simulink model "simulink_flightgear_control_trim_wind_5"  (R2023a)
settings: Solver=VariableStepAuto  StartTime=0  StopTime=inf  FixedStep=0.1  RelTol=1e-3
values from neighbouring files (symbols this model uses):
  model = 'simulink_flightgear_control_trim_wind_5'    [traimcode.m]
  ms2kts = 1.943844492609    (= 1.94384449261)    [Boeing747model.m]    (also in engine.m)
undefined symbols (not defined in the file or in its folder): Earth, F, Light, m, MIL, Model, Newton, Raphson, Receive, s, Send, Unit, WGS84, Wind
libraries: simulink_extras x7, aerolibconvert2 x5, simulink x4, aerolibfltsims x3, shared6dof x1, aerolibasang x1, aerolibtransform2 x1, aerolibatmos2 x1, aerolibobsolete x1, aerolibwind2 x1
(part 1 of 2)
settings Model: Creator=11759  LastModifiedBy=11759
settings SolverCC: ZeroCrossControl=DisableAll  ZeroCrossAlgorithm=Adaptive  EnableFixedStepZeroCrossing=on
settings DataIOCC: ExternalInput=getinputstruct(report2)  InitialState=getstatestruct(report2)  SaveFormat=StructureWithTime
settings OptimizationCC: BlockReduction=off  OptimizeBlockIOStorage=off  BufferReuse=off
settings DebuggingCC: AlgebraicLoopMsg=none  IgnoredZcDiagnostic=none
settings ModelReferenceCC: EnableRefExpFcnMdlSchedulingChecks=on
settings ExplorerConfigSet: SimMechanicsOpenEditorOnUpdate=off

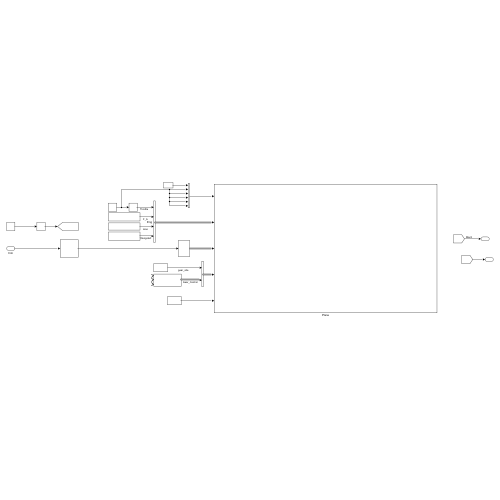
[thumbnail: Simulink's stored preview of the top-level diagram]
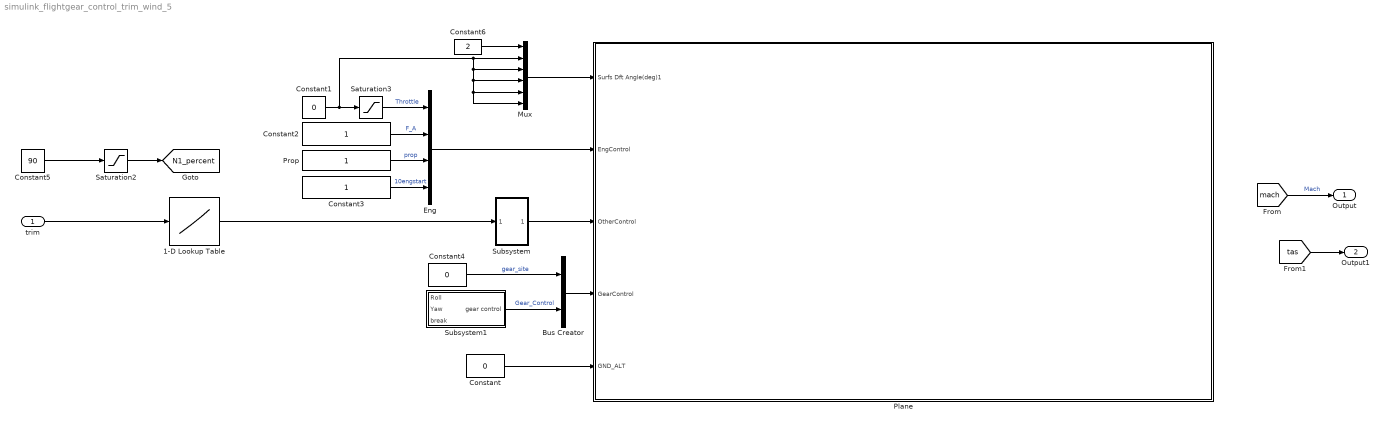
== system simulink_flightgear_control_trim_wind_5 ==
  trim : Inport
  1-D Lookup Table : Lookup_n-D  NumberOfTableDimensions=1  BreakpointsForDimension1=[-1 0 1]  Table=[-10 0 10]  InternalRulePriority=Speed  RndMeth=Simplest
  Bus Creator : BusCreator  Inputs=2
  Constant : Constant  Value=0
  Constant1 : Constant  Value=0
  Constant2 : Constant
  Constant3 : Constant
  Constant4 : Constant  Value=0
  Constant5 : Constant  Value=90
  Constant6 : Constant  Value=2
  Eng : BusCreator  Inputs=4
  Mux : Mux  Inputs=6
  Plane : Subsystem
      mask Display: image('$imagefile'); % 使用工具条上的 "编辑图像" 进行更改。
  Prop : Constant
  Saturation2 : Saturate  UpperLimit=110  LowerLimit=60
  Saturation3 : Saturate  UpperLimit=1  LowerLimit=0
  Subsystem : Subsystem
  Subsystem1 : Subsystem
  Output : Outport
  Output1 : Outport  Port=2
  tag scope: N1_percent=global
  wires:
  Mux/1 -> Plane/1(Surfs Dft Angle(deg)1)
  Constant/1 -> Plane/5(GND_ALT)
  Constant1/1 -> Mux/6, Mux/5, Mux/4, Mux/3, Mux/2, Saturation3/1
  Subsystem/1(Out1) -> Plane/3(OtherControl)
  Constant3/1 -> Eng/4  "10engstart"
  Prop/1 -> Eng/3  "prop"
  Subsystem1/1(gear control) -> Bus Creator/2  "Gear_Control"
  Constant2/1 -> Eng/2  "F_A"
  Saturation3/1 -> Eng/1  "Throttle"
  Eng/1 -> Plane/2(EngControl)
  Constant4/1 -> Bus Creator/1  "gear_site"
  Bus Creator/1 -> Plane/4(GearControl)
  Constant6/1 -> Mux/1
  Saturation2/1 -> [N1_percent]
  trim/1 -> 1-D Lookup Table/1
  1-D Lookup Table/1 -> Subsystem/1(In1)
  Constant5/1 -> Saturation2/1
  [mach] -> Output/1  "Mach"
  [tas] -> Output1/1

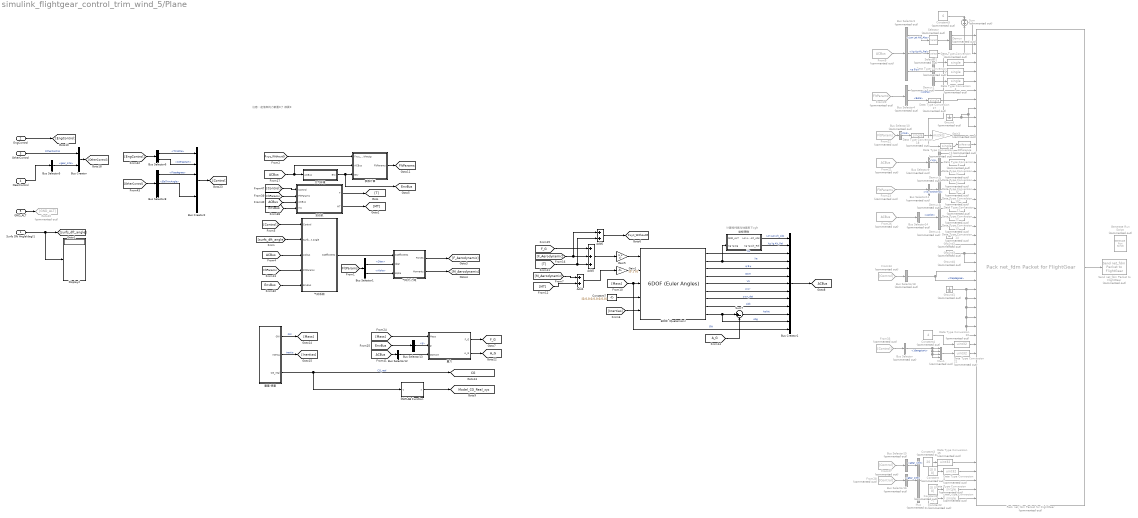
== system simulink_flightgear_control_trim_wind_5/Plane ==
  note: 注意：起落架的力都置0了
      | 襟翼0
  note: 计算经纬高与地面系下xyh
  Surfs Dft Angle(deg)1 : Inport
  EngControl : Inport  Port=2
  OtherControl : Inport  Port=3
  GearControl : Inport  Port=4
  GND_ALT : Inport  Port=5
  6DOF (Quaternion) : shared6dof/6DOF (Euler Angles)  units=Metric (MKS)  mtype=Custom Variable  rep=Euler Angles  xme_0=[0, 0, -Model.Init.Alt_Abs]  Vm_0=[Model.Init.u, Model.Init.v, Model.Init.w]  eul_0=[Model.Init.Roll, Model.Init.Pitch, Model.Init.Heading]  pm_0=[Model.Init.p, Model.Init.q, Model.Init.r]  mass_0=model.mass  mass_e=0  mass_f=0  inertia=[model.Ix -model.Ixy -model.Izx; -model.Ixy model.Iy -model.Iyz; -model.Izx -model.Iyz model.Iz]  inertia_e=eye(3)  inertia_f=eye(3)  k_quat=1.0  vre_flag=off  abi_flag=on  aMode=aMode  xme_statename=''  Vm_statename=''  eul_statename=''  quat_statename=''  pm_statename=''  mass_statename=''
  Add4 : Sum
  Add5 : Sum  Inputs=+++
  Add6 : Sum
  Bus Creator : BusCreator  Inputs=2
  Bus Creator1 : BusCreator  Inputs=13
  Bus Creator2 : BusCreator  Inputs=6
  Bus Selector : BusSelector  Commented=on  OutputSignals=10engstart
  Bus Selector1 : BusSelector  OutputSignals=Qbar,Alpha
  Bus Selector10 : BusSelector  Commented=on  OutputSignals=CAS
  Bus Selector11 : BusSelector  Commented=on  OutputSignals=Vb_WithWind
  Bus Selector12 : BusSelector  OutputSignals=DCM  OutputAsBus=on
  Bus Selector13 : BusSelector  OutputSignals=g
  Bus Selector14 : BusSelector  Commented=on  OutputSignals=Apilot
  Bus Selector15 : BusSelector  Commented=on  OutputSignals=gear_site
  Bus Selector16 : BusSelector  Commented=on  OutputSignals=gear_site
  Bus Selector18 : BusSelector  Commented=on  OutputSignals=Flapdegree
  Bus Selector3 : BusSelector  Commented=on  OutputSignals=Lon Lat Alt_Abs,Xg Yg Alt_Rel,φ θ ψ
  Bus Selector4 : BusSelector  Commented=on  OutputSignals=Alpha,Beta
  Bus Selector5 : BusSelector  OutputSignals=gear_site
  Bus Selector6 : BusSelector  OutputSignals=Throttle,10engstart
  Bus Selector8 : BusSelector  OutputSignals=OtherControl.Flapdegree,OtherControl.EleTrimAngle,OtherControl.SpoilerPercent
  Bus Selector9 : BusSelector  Commented=on  OutputSignals=Vg
  Constant : Constant  Commented=on  Value=[0 0 0]
  Constant1 : Constant  Commented=on  Value=[0 0 0]
  Constant2 : Constant  Commented=on  Value=[0 0 0]
  Constant3 : Constant  Commented=on  Value=20
  Constant4 : Constant  Commented=on  Value=4
  Constant5 : Constant  Commented=on  Value=6
  Constant7 : Constant  Value=[0,0,0;0,0,0;0,0,0]
  Data Type Conversion{,1..7,9..14,17..19} (17 alike) : DataTypeConversion  Commented=on  OutDataTypeStr=single  SaturateOnIntegerOverflow=off  RndMeth=Floor
  Data Type Conversion{8,15,20..21} (4 alike) : DataTypeConversion  Commented=on  OutDataTypeStr=uint32  SaturateOnIntegerOverflow=off  RndMeth=Floor
  Demux : Demux  Commented=on  Outputs=2
  Demux{1..4} (4 alike) : Demux  Commented=on  Outputs=3
  Difference : simulink/Discrete/Difference  Commented=on  ICPrevInput=0.0  OutMin=[]  OutMax=[]  OutDataType=fixdt(1, 16)  OutScaling=2^-10  DoSatur=off
  Display2 : Display
  From20 : From  Commented=on  GotoTag=FltParams  TagVisibility=global
  From21 : From  Commented=on  GotoTag=ACBus  TagVisibility=global
  From22 : From  Commented=on  GotoTag=FltParams  TagVisibility=global
  From23 : From  Commented=on  GotoTag=FltParams  TagVisibility=global
  From26 : From  Commented=on  GotoTag=ACBus  TagVisibility=global
  From{27..28,33..34} (4 alike) : From  Commented=on  GotoTag=Control
  From9 : From  Commented=on  GotoTag=ACBus  TagVisibility=global
  Gain1 : Gain  Gain=[0 1 0]'
  Gain3 : Gain  Commented=on  Gain=ms2kts
  Gain5 : Gain  Gain=[1 0 1]'
  Generate Run Script : aerolibfltsims/Generate Run Script  Commented=on  Architecture=Win64  dataFlow=Send-Receive  GeometryModelName=747-400  AirportId=KSFO  RunwayId=10L  InitialAltitude=1000  InitialHeading=113  OffsetDistance=4.72  OffsetAzimuth=0  InstallScenery=off  DisableShaders=on  OriginAddress=127.0.0.1  DestinationPort=5502  OriginPort=5505  LocalAddress=127.0.0.1  OutputFileName=runfg.bat  FlightGearBaseDirectory=E:\flightgear\FlightGear 2020.3
  Goto20 : Goto  Commented=on  GotoTag=GND_ALT
  Ground{,1..4} (5 alike) : Ground  Commented=on
  MATLAB Function : MATLAB Function  TreatAsAtomicUnit=on
  Mux : Mux  Commented=on  Inputs=3
  Mux1 : Mux  Commented=on
  Pack net_fdm Packet for FlightGear : aerolibfltsims/Pack net_fdm Packet for FlightGear  Commented=on  FlightGearVersion=v2019.1  ShowPositionAttitudeInputs=on  ShowVelocityAccelerationInputs=on  ShowControlSurfacePositionInputs=on  ShowEngineFuelInputs=on  ShowLandingGearInputs=on  ShowEnvironmentInputs=off  SampleTime=0.1  packetVersion=24
  Selector : Selector  Commented=on  InputPortWidth=3  IndexOptions=Index vector (dialog)  Indices=[1 2]  OutputSizes=1
  Selector1 : Selector  Commented=on  InputPortWidth=3  IndexOptions=Index vector (dialog)  Indices=[3]  OutputSizes=1
  Send net_fdm Packet to FlightGear : aerolibfltsims/Send net_fdm Packet to FlightGear  Commented=on  DestinationIpAddress=127.0.0.1  DestinationPort=5502  LocalIpPort=-1  varLen=off  SampleTime=0.1
  Sum : Sum  Commented=on
  Sum7 : Sum  Inputs=|+-
  参数计算 : Subsystem
  发动机 : Subsystem
  坐标转换 : Subsystem
  大气环境 : Subsystem
  气动力/力矩 : Subsystem
  气动系数 : Subsystem
  "重力 " : Subsystem
  重量/惯量 : Subsystem
  tag scope: ACBus=global, A_G=global, CG=global, EnvBus=global, F_G=global, FltParams=global, Fxyz_WithoutG=global, Model_CG_Real_xyz=global
  wires:
  EngControl/1 -> [EngControl]
  OtherControl/1 -> Bus Creator/1  "OtherControl"
  Bus Creator/1 -> [OtherControl]
  GearControl/1 -> Bus Selector5/1
  Bus Selector5/1 -> Bus Creator/2  "<gear_site>"
  GND_ALT/1 -> Goto20/1
  Bus Selector6/1 -> Bus Creator2/1  "<Throttle>"
  Bus Creator2/1 -> [Control]
  Bus Selector8/1 -> Bus Creator2/3  "<Flapdegree>"
  Bus Selector6/2 -> Bus Creator2/2  "<10engstart>"
  [EngControl] -> Bus Selector6/1
  [OtherControl] -> Bus Selector8/1
  Surfs Dft Angle(deg)1/1 -> [surfs_dft_angle], Display2/1
  [ACBus] -> 气动系数/3(ACbus)
  [Control] -> 气动系数/1(Control)
  [FltParams] -> 气动系数/4(FltParams)
  [surfs_dft_angle] -> 气动系数/2(Surfs Dft Angle)
  Bus Selector8/2 -> Bus Creator2/5  "<EleTrimAngle>"
  [EnvBus] -> 气动系数/5(EnvBus)
  MATLAB Function/1(y) -> [Model_CG_Real_xyz]
  重量/惯量/3(CG_real) -> MATLAB Function/1(u), [CG]  "CG_real"
  重量/惯量/1(GW) -> [Mass]  "GW"
  重量/惯量/2(Inertia) -> [Inertias]  "Inertia"
  发动机/1(T) -> [T]
  [ACBus] -> 发动机/3(ACBus)
  [Control] -> 发动机/1(Control)
  [ACBus] -> 大气环境/1(ACBus), 参数计算/2(ACBus)
  [EnvBus] -> 发动机/4(In1)
  大气环境/1(Env) -> [EnvBus], 参数计算/3(Env)
  [Fxyz_WithoutG] -> 参数计算/1(Fxyz_withoutg)
  发动机/2(MT) -> [MT]
  参数计算/1(FltParams) -> [FltParams]
  [FltParams] -> 发动机/2(FltParams)
  [FltParams] -> Bus Selector1/1
  Bus Selector1/1 -> 气动力/力矩/2(qbar)  "<Qbar>"
  Bus Selector1/2 -> 气动力/力矩/3(alpha)  "<Alpha>"
  气动系数/1(Coefficients) -> 气动力/力矩/1(Coefficients)
  气动力/力矩/2(Moments) -> [M_Aerodynamic]
  气动力/力矩/1(Forces) -> [F_Aerodynamic]
  "重力 "/1(F_G) -> [F_G]
  Bus Selector13/1 -> "重力 "/2(g)  "<g>"
  [EnvBus] -> Bus Selector13/1
  Bus Selector12/1 -> "重力 "/3(DCMwe)
  [ACBus] -> Bus Selector12/1
  [Mass] -> "重力 "/1(Mass)
  "重力 "/2(A_G) -> [A_G]
  Bus Selector4/1 -> Pack net_fdm Packet for FlightGear/7  "<Alpha>"
  Bus Selector4/2 -> Data Type Conversion17/1  "<Beta>"
  Data Type Conversion13/1 -> Pack net_fdm Packet for FlightGear/21
  Bus Selector9/1 -> Demux2/1  "<Vg>"
  Demux1/3 -> Data Type Conversion2/1
  Demux2/3 -> Data Type Conversion5/1
  Data Type Conversion21/1 -> Pack net_fdm Packet for FlightGear/36
  Constant2/1 -> Data Type Conversion7/1
  Demux1/1 -> Data Type Conversion/1
  Demux4/1 -> Data Type Conversion12/1
  Demux2/1 -> Data Type Conversion3/1
  Selector/1 -> Demux/1
  Demux/2 -> Pack net_fdm Packet for FlightGear/2
  Data Type Conversion12/1 -> Pack net_fdm Packet for FlightGear/20
  Data Type Conversion4/1 -> Pack net_fdm Packet for FlightGear/15
  Bus Selector3/2 -> Selector1/1  "<Xg Yg Alt_Rel>"
  Ground2/1 -> Pack net_fdm Packet for FlightGear/23
  Demux3/1 -> Data Type Conversion9/1
  Data Type Conversion10/1 -> Pack net_fdm Packet for FlightGear/18
  Data Type Conversion20/1 -> Pack net_fdm Packet for FlightGear/35
  From9/1 -> Bus Selector3/1
  Data Type Conversion15/1 -> Pack net_fdm Packet for FlightGear/48
  Demux4/2 -> Data Type Conversion13/1
  Bus Selector10/1 -> Data Type Conversion18/1  "<CAS>"
  Bus Selector16/1 -> Mux/2  "<gear_site>"
  Difference/1 -> Pack net_fdm Packet for FlightGear/13
  Bus Selector11/1 -> Demux3/1  "<Vb_WithWind>"
  Mux1/1 -> Data Type Conversion21/1
  Demux3/2 -> Data Type Conversion10/1
  Constant5/1 -> Sum/1
  Data Type Conversion1/1 -> Pack net_fdm Packet for FlightGear/5
  From21/1 -> Bus Selector9/1
  Data Type Conversion14/1 -> Pack net_fdm Packet for FlightGear/22
  Data Type Conversion19/1 -> Difference/1
  Mux/1 -> Pack net_fdm Packet for FlightGear/50
  Data Type Conversion18/1 -> Gain3/1
  From27/1 -> Bus Selector15/1
  Demux2/2 -> Data Type Conversion4/1
  Data Type Conversion7/1 -> Pack net_fdm Packet for FlightGear/52
  From33/1 -> Bus Selector/1
  Constant4/1 -> Data Type Conversion20/1
  From34/1 -> Bus Selector18/1
  Data Type Conversion6/1 -> Pack net_fdm Packet for FlightGear/51
  Constant/1 -> Data Type Conversion8/1
  Ground1/1 -> Pack net_fdm Packet for FlightGear/34, Pack net_fdm Packet for FlightGear/33, Pack net_fdm Packet for FlightGear/32, Pack net_fdm Packet for FlightGear/31, Pack net_fdm Packet for FlightGear/30, Pack net_fdm Packet for FlightGear/29
  From20/1 -> Bus Selector4/1
  Bus Selector14/1 -> Demux4/1  "<Apilot>"
  Data Type Conversion9/1 -> Pack net_fdm Packet for FlightGear/17
  Constant1/1 -> Data Type Conversion6/1
  Demux3/3 -> Data Type Conversion11/1
  Bus Selector3/3 -> Demux1/1  "<φ θ ψ>"
  Data Type Conversion8/1 -> Pack net_fdm Packet for FlightGear/49
  Demux4/3 -> Data Type Conversion14/1
  Bus Selector3/1 -> Selector/1  "<Lon Lat Alt_Abs>"
  Data Type Conversion2/1 -> Pack net_fdm Packet for FlightGear/6
  Bus Selector/1 -> Mux1/4, Mux1/3, Mux1/2, Mux1/1  "<10engstart>"
  Gain3/1 -> Pack net_fdm Packet for FlightGear/12
  Constant3/1 -> Data Type Conversion15/1
  Data Type Conversion5/1 -> Pack net_fdm Packet for FlightGear/16
  Selector1/1 -> Sum/2, Data Type Conversion19/1
  From22/1 -> Bus Selector10/1
  Bus Selector18/1 -> Pack net_fdm Packet for FlightGear/28, Pack net_fdm Packet for FlightGear/27  "<Flapdegree>"
  Bus Selector15/1 -> Mux/1  "<gear_site>"
  Demux/1 -> Pack net_fdm Packet for FlightGear/1
  Ground4/1 -> Pack net_fdm Packet for FlightGear/26, Pack net_fdm Packet for FlightGear/25
  Pack net_fdm Packet for FlightGear/1 -> Send net_fdm Packet to FlightGear/1
  Data Type Conversion11/1 -> Pack net_fdm Packet for FlightGear/19
  From28/1 -> Bus Selector16/1
  Data Type Conversion/1 -> Pack net_fdm Packet for FlightGear/4
  Sum/1 -> Pack net_fdm Packet for FlightGear/3
  Data Type Conversion17/1 -> Pack net_fdm Packet for FlightGear/8
  From23/1 -> Bus Selector11/1
  Ground3/1 -> Pack net_fdm Packet for FlightGear/24
  Demux1/2 -> Data Type Conversion1/1
  From26/1 -> Bus Selector14/1
  Ground/1 -> Pack net_fdm Packet for FlightGear/9, Pack net_fdm Packet for FlightGear/11, Pack net_fdm Packet for FlightGear/10
  Data Type Conversion3/1 -> Pack net_fdm Packet for FlightGear/14
  Sum7/1 -> Bus Creator1/11  "Apilot"
  6DOF (Quaternion)/1 -> Bus Creator1/3  "Vg"
  6DOF (Quaternion)/7 -> Bus Creator1/9  "p q r_dot"
  坐标转换/1(Lon Lat Alt_Abs) -> Bus Creator1/1  "Lon Lat Alt_Abs"
  坐标转换/2(Xg Yg Alt_Rel) -> Bus Creator1/2  "Xg Yg Alt_Rel"
  6DOF (Quaternion)/3 -> Bus Creator1/5  "φ θ ψ"
  [A_G] -> Sum7/2
  6DOF (Quaternion)/8 -> Bus Creator1/10  "Abb"
  6DOF (Quaternion)/5 -> Bus Creator1/7  "Vb"
  Bus Creator1/1 -> [ACBus]
  6DOF (Quaternion)/6 -> Bus Creator1/8  "p q r"
  6DOF (Quaternion)/4 -> Bus Creator1/6  "DCM"
  [Mass] -> Bus Creator1/13, 6DOF (Quaternion)/3  "GW"
  6DOF (Quaternion)/2 -> 坐标转换/2(Xg Yg Zg), Bus Creator1/4  "Xe"
  6DOF (Quaternion)/9 -> Sum7/1, Bus Creator1/12  "Abg"
  Add6/1 -> [Fxyz_WithoutG]
  [MT] -> Add4/2
  [M_Aerodynamic] -> Add4/1
  Add5/1 -> Gain5/1
  [F_Aerodynamic] -> Add5/2, Add6/1
  [F_G] -> Add5/1
  [T] -> Add5/3, Add6/2
  [Inertias] -> 6DOF (Quaternion)/5
  Constant7/1 -> 6DOF (Quaternion)/4
  Add4/1 -> Gain1/1
  Gain5/1 -> 6DOF (Quaternion)/1
  Gain1/1 -> 6DOF (Quaternion)/2

== system simulink_flightgear_control_trim_wind_5/Subsystem ==
  In1 : Inport
  Bus Creator : BusCreator  Inputs=4
  Constant2 : Constant  Value=0
  Constant4 : Constant  Value=0
  Data Type Conversion13 : DataTypeConversion  OutDataTypeStr=single  SaturateOnIntegerOverflow=off  RndMeth=Floor
  Gain : Gain
  Out1 : Outport
  wires:
  Constant4/1 -> Bus Creator/2  "SpoilerPercent"
  Data Type Conversion13/1 -> Bus Creator/1  "Flapdegree"
  Gain/1 -> Bus Creator/4  "EleTrimAngle"
  Constant2/1 -> Bus Creator/3  "RudTrimAngle"
  Bus Creator/1 -> Out1/1
  In1/1 -> Gain/1

== system simulink_flightgear_control_trim_wind_5/Subsystem1 ==
  Roll : Inport
  Yaw : Inport  Port=2
  break : Inport  Port=3
  Bus Creator : BusCreator  Inputs=3
  Constant : Constant  Value=0
  Constant1 : Constant  Value=0
  Constant2 : Constant  Value=0
  Gain4 : Gain
  Gain5 : Gain  Gain=-1
  Gain6 : Gain  Gain=0
  Mux1 : Mux  Inputs=3
  Mux2 : Mux  Inputs=3
  Saturation4 : Saturate  UpperLimit=1  LowerLimit=0
  Saturation5 : Saturate  UpperLimit=0  LowerLimit=-1
  Sum : Sum  Inputs=-+|
  Sum1 : Sum  Inputs=++|
  gear control : Outport
  wires:
  Constant/1 -> Mux1/1
  break/1 -> Sum1/1, Sum/1
  Constant2/1 -> Bus Creator/3  "Retract"
  Yaw/1 -> Gain6/1
  Sum/1 -> Saturation5/1
  Mux1/1 -> Bus Creator/1  "Brake"
  Gain5/1 -> Mux1/2  "Lbrake"
  Gain4/1 -> Mux1/3  "Rbrake"
  Mux2/1 -> Bus Creator/2  "Steering"
  Sum1/1 -> Saturation4/1
  Constant1/1 -> Mux2/3, Mux2/2
  Gain6/1 -> Mux2/1
  Roll/1 -> Sum1/2, Sum/2
  Saturation5/1 -> Gain5/1
  Saturation4/1 -> Gain4/1
  Bus Creator/1 -> gear control/1

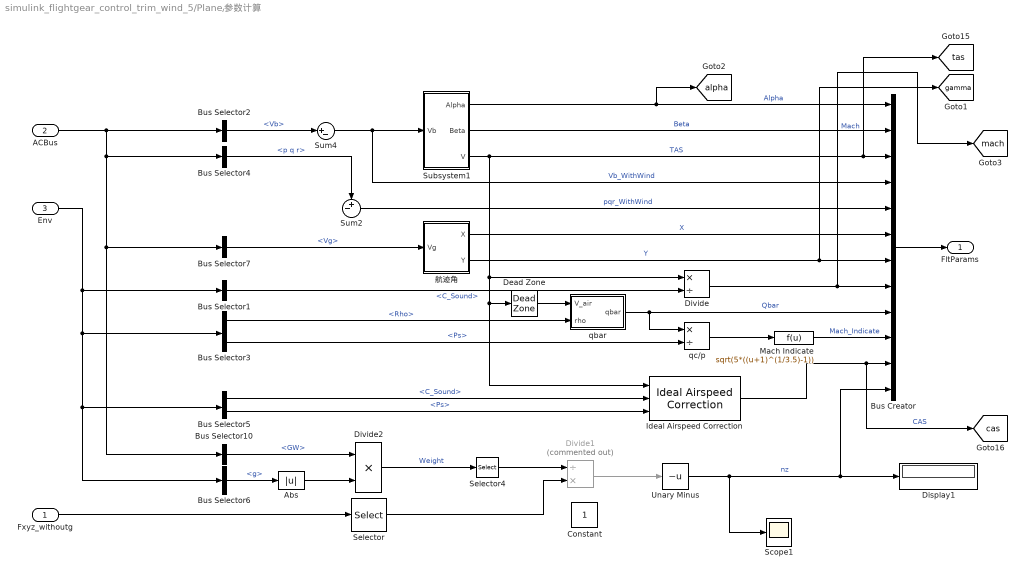
== system simulink_flightgear_control_trim_wind_5/Plane/参数计算 ==
  Fxyz_withoutg : Inport
  ACBus : Inport  Port=2
  Env : Inport  Port=3
  Abs : Abs  SaturateOnIntegerOverflow=off
  Bus Creator : BusCreator  Inputs=12
  Bus Selector1 : BusSelector  OutputSignals=C_Sound
  Bus Selector10 : BusSelector  OutputSignals=GW
  Bus Selector2 : BusSelector  OutputSignals=Vb
  Bus Selector3 : BusSelector  OutputSignals=Rho,Ps
  Bus Selector4 : BusSelector  OutputSignals=p q r
  Bus Selector5 : BusSelector  OutputSignals=C_Sound,Ps
  Bus Selector6 : BusSelector  OutputSignals=g
  Bus Selector7 : BusSelector  OutputSignals=Vg
  Constant : Constant
  Dead Zone : DeadZone  LowerValue=-0.05  UpperValue=0.05
  Display1 : Display
  Divide : Product  Inputs=*/
  Divide1 : Product  Commented=on  Inputs=/*
  Divide2 : Product  Inputs=**
  Ideal Airspeed Correction : aerolibasang/Ideal Airspeed Correction  units=Metric (MKS)  vel_in=TAS  vel_out_tas=CAS  vel_out_eas=TAS  vel_out_cas=TAS  method=Table Lookup  SubOnly=off  action=None
  Mach Indicate : Fcn  Expr=sqrt(5*((u+1)^(1/3.5)-1))
  Scope1 : Scope
  Selector : Selector  InputPortWidth=3  IndexOptions=Index vector (dialog)  Indices=[3]  OutputSizes=1
  Selector4 : Selector  InputPortWidth=3  IndexOptions=Index vector (dialog)  Indices=[3]  OutputSizes=1
  Subsystem1 : Subsystem
  Sum2 : Sum  Inputs=+-|  InputSameDT=on  SaturateOnIntegerOverflow=on  OutDataTypeStr=Inherit: Same as first input
  Sum4 : Sum  Inputs=|+-  InputSameDT=on  SaturateOnIntegerOverflow=on  OutDataTypeStr=Inherit: Same as first input
  Unary Minus : UnaryMinus
  qbar : Subsystem
  qc/p : Product  Inputs=*/
  航迹角 : Subsystem
  FltParams : Outport  VectorParamsAs1DForOutWhenUnconnected=off
  tag scope: alpha=global, cas=global, gamma=global, mach=global, tas=global
  wires:
  Bus Selector7/1 -> 航迹角/1(Vg)  "<Vg>"
  ACBus/1 -> Bus Selector2/1, Bus Selector4/1, Bus Selector10/1, Bus Selector7/1
  航迹角/2(Y) -> [gamma], Bus Creator/7  "Y"
  航迹角/1(X) -> Bus Creator/6  "X"
  Bus Selector2/1 -> Sum4/1  "<Vb>"
  Bus Selector3/2 -> qc/p/2  "<Ps>"
  Bus Selector3/1 -> qbar/2(rho)  "<Rho>"
  Bus Selector4/1 -> Sum2/1  "<p q r>"
  Bus Creator/1 -> FltParams/1
  Subsystem1/2(Beta) -> Bus Creator/2  "Beta"
  Subsystem1/1(Alpha) -> [alpha], Bus Creator/1  "Alpha"
  qbar/1(qbar) -> qc/p/1, Bus Creator/9  "Qbar"
  qc/p/1 -> Mach Indicate/1
  Mach Indicate/1 -> Bus Creator/10  "Mach_Indicate"
  Divide/1 -> [mach], Bus Creator/8  "Mach"
  Bus Selector1/1 -> Divide/2  "<C_Sound>"
  Sum2/1 -> Bus Creator/5  "pqr_WithWind"
  Sum4/1 -> Subsystem1/1(Vb), Bus Creator/4  "Vb_WithWind"
  Subsystem1/3(V) -> Divide/1, Ideal Airspeed Correction/1, Dead Zone/1, [tas], Bus Creator/3  "TAS"
  Env/1 -> Bus Selector6/1, Bus Selector5/1, Bus Selector3/1, Bus Selector1/1
  Bus Selector5/2 -> Ideal Airspeed Correction/3  "<Ps>"
  Bus Selector5/1 -> Ideal Airspeed Correction/2  "<C_Sound>"
  Ideal Airspeed Correction/1 -> [cas], Bus Creator/11  "CAS"
  Dead Zone/1 -> qbar/1(V_air)
  Fxyz_withoutg/1 -> Selector/1
  Bus Selector6/1 -> Abs/1  "<g>"
  Bus Selector10/1 -> Divide2/1  "<GW>"
  Abs/1 -> Divide2/2
  Divide2/1 -> Selector4/1  "Weight"
  Divide1/1 -> Unary Minus/1
  Selector/1 -> Divide1/2
  Selector4/1 -> Divide1/1
  Unary Minus/1 -> Scope1/1, Bus Creator/12, Display1/1  "nz"

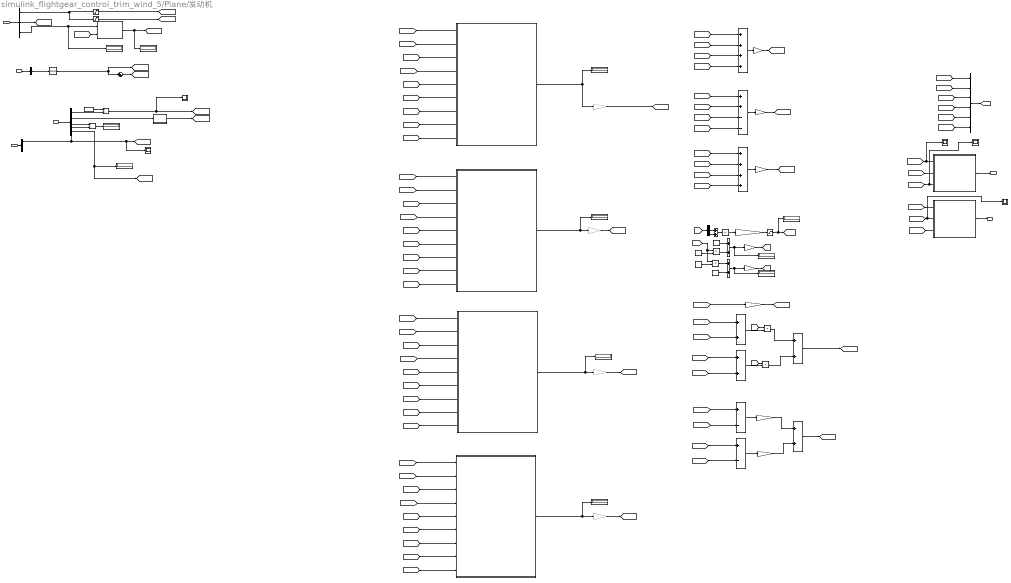
== system simulink_flightgear_control_trim_wind_5/Plane/发动机 ==
  note: 1号为最左边
  note: 华氏温度
  Control : Inport
  FltParams : Inport  Port=2
  ACBus : Inport  Port=3
  In1 : Inport  Port=4
  Abs4 : Abs  SaturateOnIntegerOverflow=off
  Bus Creator : BusCreator  Inputs=6
  Bus Selector : BusSelector  OutputSignals=Throttle,10engstart,Flapdegree
  Bus Selector1 : BusSelector  OutputSignals=Lon Lat Alt_Abs
  Bus Selector2 : BusSelector  OutputSignals=Mach,CAS,TAS
  Bus Selector5 : BusSelector  OutputSignals=Ps,Ts,C_Sound,Rho
  Constant4 : Constant  Value=1.9
  Constant7 : Constant  Value=-5.4
  Constant8 : Constant  Value=5.4
  Constant9 : Constant  Value=14.6
  Demux5 : Demux  Outputs=3
  Display{,1..2,4..8,10..12} (11 alike) : Display
  Divide1 : Product  Inputs=/*
  Divide2 : Product  Inputs=/*
  Gain : Gain  Gain=0.0349
  Gain1 : Gain  Gain=-0.0436
  Gain16 : Gain  Gain=39.370078740157/36
  Gain18 : Gain  Gain=Unit.ft2m
  Gain19 : Gain  Gain=Unit.ft2m
  Gain2 : Gain  Gain=21.15312
  Gain3 : Gain  Gain=12.07008
  Gain4 : Gain  Gain=0.436
  Gain{5..6,8..9} (4 alike) : Gain  Commented=through  Gain=1.1
  Gain7 : Gain
  MATLAB Function : MATLAB Function  TreatAsAtomicUnit=on
  MATLAB Function1 : MATLAB Function  TreatAsAtomicUnit=on
  MATLAB Function2 : MATLAB Function  TreatAsAtomicUnit=on
  MATLAB Function4 : MATLAB Function  TreatAsAtomicUnit=on
  Product{2..5} (4 alike) : Product
  Saturation10 : Saturate  UpperLimit=1  LowerLimit=-1
  Saturation2 : Saturate  UpperLimit=1  LowerLimit=0
  Saturation8 : Saturate  UpperLimit=1  LowerLimit=-1
  Scope{,1..3,5} (5 alike) : Scope
  Selector : Selector  InputPortWidth=3  IndexOptions=Index vector (dialog)  Indices=[ 3]  OutputSizes=1
  Subsystem : Subsystem
  Subsystem1 : Subsystem
  Subsystem2 : Subsystem
  Subsystem3 : Subsystem
  Sum : Sum  Inputs=++++
  Sum1 : Sum  Inputs=++--
  Sum{5..8,13..15} (7 alike) : Sum
  Sum16 : Sum  Inputs=|++
  Sum2 : Sum  Inputs=++++
  Sum3 : Sum  Inputs=+-
  Sum4 : Sum  Inputs=+-
  p1 : Constant  Value=101325
  T : Outport  VectorParamsAs1DForOutWhenUnconnected=off
  MT : Outport  Port=2  VectorParamsAs1DForOutWhenUnconnected=off
  tag scope: Engine=global, rho=global
  wires:
  [gear_hg] -> Subsystem/5(In5)
  Gain2/1 -> Sum5/1
  [FN_1] -> Sum1/1
  [FN_2] -> Sum4/1
  [gear_position] -> Subsystem/4(In4)
  [FN_3] -> Sum4/2
  [FN_1] -> Sum6/1
  [FN_2] -> Sum/2
  Sum6/1 -> Product4/2
  Gain1/1 -> [T_z]
  [deltaAM] -> Subsystem/8(In8)
  [FN_4] -> Sum3/2
  Sum4/1 -> Gain3/1
  [FN_2] -> Sum2/2
  [FN_1] -> Sum/1
  [FN_2] -> Sum1/2
  [FN_2] -> Sum7/1
  [high] -> Subsystem/7(In7)
  [FN_3] -> Sum7/2
  [mach] -> Subsystem/6(In6)
  Sum3/1 -> Gain2/1
  [FN_4] -> Sum6/2
  [FN_3] -> Sum1/3
  [FN_4] -> Sum/4
  [throttleangle] -> Subsystem/1(In1)
  [FN_1] -> Sum3/1
  Sum7/1 -> Product5/2
  [FN_3] -> Sum/3
  Product4/1 -> Sum8/1
  Sum2/1 -> Gain1/1
  [TAM] -> Subsystem/2(In2)
  Gain/1 -> [T_y]
  [FN_3] -> Sum2/3
  [FN_4] -> Sum1/4
  Gain3/1 -> Sum5/2
  [site] -> Subsystem/3(In3)
  Sum/1 -> Gain7/1
  [FN_1] -> Sum2/1
  [FN_4] -> Sum2/4
  Sum1/1 -> Gain/1
  Control/1 -> Bus Selector/1
  ACBus/1 -> Bus Selector1/1
  FltParams/1 -> Bus Selector2/1
  [T_x] -> Scope/1, MATLAB Function/1(x)
  [T_y] -> MATLAB Function/2(y)
  [T_z] -> Scope3/1, MATLAB Function/3(z)
  MATLAB Function/1(T) -> T/1
  [N_T] -> MATLAB Function1/3(z)
  [M_T] -> Scope5/1, MATLAB Function1/2(y)
  [L_T] -> MATLAB Function1/1(x)
  MATLAB Function1/1(MT) -> MT/1
  [N_T] -> Bus Creator/6
  [M_T] -> Bus Creator/5
  [L_T] -> Bus Creator/4
  [T_z] -> Bus Creator/3
  [T_y] -> Bus Creator/2
  [T_x] -> Bus Creator/1
  Bus Creator/1 -> [Engine]
  Bus Selector/1 -> Saturation8/1, Saturation10/1  "<Throttle>"
  [mach] -> MATLAB Function2/2(ma)
  Saturation8/1 -> [throttleangle]
  MATLAB Function2/1(site) -> Display1/1, [site]
  Saturation10/1 -> [throttleangle2]
  Bus Selector/2 -> [power_on]  "<10engstart>"
  Selector/1 -> Sum16/1, [gear_hg]
  Bus Selector1/1 -> Selector/1  "<Lon Lat Alt_Abs>"
  Bus Selector2/1 -> Scope2/1, [mach], Divide2/2  "<Mach>"
  Bus Selector/3 -> MATLAB Function2/1(flap), Display/1  "<Flapdegree>"
  Sum8/1 -> [M_T]
  [power_on] -> Subsystem/9(In9)
  [high] -> Subsystem1/7(In7)
  [site] -> Subsystem1/3(In3)
  [deltaAM] -> Subsystem1/8(In8)
  [mach] -> Subsystem1/6(In6)
  [gear_position] -> Subsystem1/4(In4)
  [gear_hg] -> Subsystem1/5(In5)
  [throttleangle] -> Subsystem1/1(In1)
  [power_on] -> Subsystem1/9(In9)
  [TAM] -> Subsystem1/2(In2)
  [high] -> Subsystem2/7(In7)
  [site] -> Subsystem2/3(In3)
  [deltaAM] -> Subsystem2/8(In8)
  [mach] -> Subsystem2/6(In6)
  [gear_position] -> Subsystem2/4(In4)
  [gear_hg] -> Subsystem2/5(In5)
  [throttleangle2] -> Subsystem2/1(In1)
  [power_on] -> Subsystem2/9(In9)
  [TAM] -> Subsystem2/2(In2)
  [high] -> Subsystem3/7(In7)
  [site] -> Subsystem3/3(In3)
  [deltaAM] -> Subsystem3/8(In8)
  [mach] -> Subsystem3/6(In6)
  [gear_position] -> Subsystem3/4(In4)
  [gear_hg] -> Subsystem3/5(In5)
  [throttleangle2] -> Subsystem3/1(In1)
  [power_on] -> Subsystem3/9(In9)
  [TAM] -> Subsystem3/2(In2)
  Gain7/1 -> [T_x]
  Sum5/1 -> [N_T]
  Bus Selector5/4 -> [rho], Display5/1  "<Rho>"
  Divide2/1 -> Display4/1
  Divide1/1 -> Scope1/1, [deltaAM]
  MATLAB Function4/1(y) -> [TAM]
  Bus Selector5/2 -> MATLAB Function4/1(u)  "<Ts>"
  In1/1 -> Bus Selector5/1  "envbus"
  Abs4/1 -> Gain16/1
  Saturation2/1 -> Display6/1, [K_eepa]
  Sum13/1 -> Abs4/1
  Gain16/1 -> Saturation2/1
  Demux5/3 -> Sum13/2
  [ST] -> Demux5/1
  Demux5/2 -> Sum13/1
  Constant7/1 -> Product3/2
  Constant4/1 -> Product2/2
  Product2/1 -> Sum14/2
  Constant8/1 -> Sum14/1
  Product3/1 -> Sum15/1
  Constant9/1 -> Sum15/2
  Sum15/1 -> Display8/1, Gain19/1
  Sum14/1 -> Display7/1, Gain18/1
  [K_eepa] -> Product3/1, Product2/1
  Gain18/1 -> [Z_eo]
  Gain19/1 -> [Z_ei]
  [Z_eo] -> Product4/1
  [Z_ei] -> Product5/1
  Product5/1 -> Sum8/2
  [N_T] -> Gain4/1
  Gain4/1 -> [L_T]
  Subsystem/1(single_engine_thrust_lbf) -> Gain5/1, Display2/1
  Subsystem1/1(single_engine_thrust_lbf) -> Gain6/1, Display10/1
  Subsystem3/1(single_engine_thrust_lbf) -> Display12/1, Gain9/1
  Bus Selector5/3 -> Divide2/1  "<C_Sound>"
  p1/1 -> Divide1/1
  Bus Selector5/1 -> Divide1/2  "<Ps>"
  Sum16/1 -> [high]
  Gain5/1 -> [FN_1]
  Gain6/1 -> [FN_2]
  Subsystem2/1(single_engine_thrust_lbf) -> Display11/1, Gain8/1
  Gain9/1 -> [FN_4]
  Gain8/1 -> [FN_3]

== system simulink_flightgear_control_trim_wind_5/Plane/坐标转换 ==
  GND_ALT : Inport
  Xg Yg Zg : Inport  Port=2
  Angle Conversion : aerolibconvert2/Angle Conversion  IU=deg  OU=rad
  Flat Earth to LLA : aerolibtransform2/Flat Earth to LLA  units=Metric (MKS)  ptype=Earth (WGS84)  F=1/298.257223563  R=6378137  refPosPort=off  LL0=Model.Init.latlong  psi=0
  Mux : Mux  Inputs=2
  Mux1 : Mux  Inputs=2
  Selector : Selector  IndexMode=Zero-based  InputPortWidth=2  IndexOptions=Index vector (dialog)  Indices=[1 0]  OutputSizes=1
  Selector1 : Selector  InputPortWidth=3  IndexOptions=Index vector (dialog)  Indices=[1 2]  OutputSizes=1
  Selector2 : Selector  InputPortWidth=3  IndexOptions=Index vector (dialog)  Indices=[3]  OutputSizes=1
  Sum : Sum  Inputs=|++
  Sum1 : Sum  Inputs=|++
  xyH : Gain  Gain=[1 1 -1]  SaturateOnIntegerOverflow=on  OutDataTypeStr=Inherit: Same as input  ParamDataTypeStr=Inherit: Same as input
  Lon Lat Alt_Abs : Outport  VectorParamsAs1DForOutWhenUnconnected=off
  Xg Yg Alt_Rel : Outport  Port=2  VectorParamsAs1DForOutWhenUnconnected=off
  wires:
  Angle Conversion/1 -> Mux/1
  Selector/1 -> Angle Conversion/1
  Xg Yg Zg/1 -> xyH/1, Flat Earth to LLA/1
  Flat Earth to LLA/1 -> Selector/1
  xyH/1 -> Selector2/1, Selector1/1
  Mux1/1 -> Xg Yg Alt_Rel/1
  Selector1/1 -> Mux1/1
  Mux/1 -> Lon Lat Alt_Abs/1
  Selector2/1 -> Sum1/1
  GND_ALT/1 -> Flat Earth to LLA/2
  Flat Earth to LLA/2 -> Sum/1
  Sum1/1 -> Mux/2
  Sum/1 -> Mux1/2

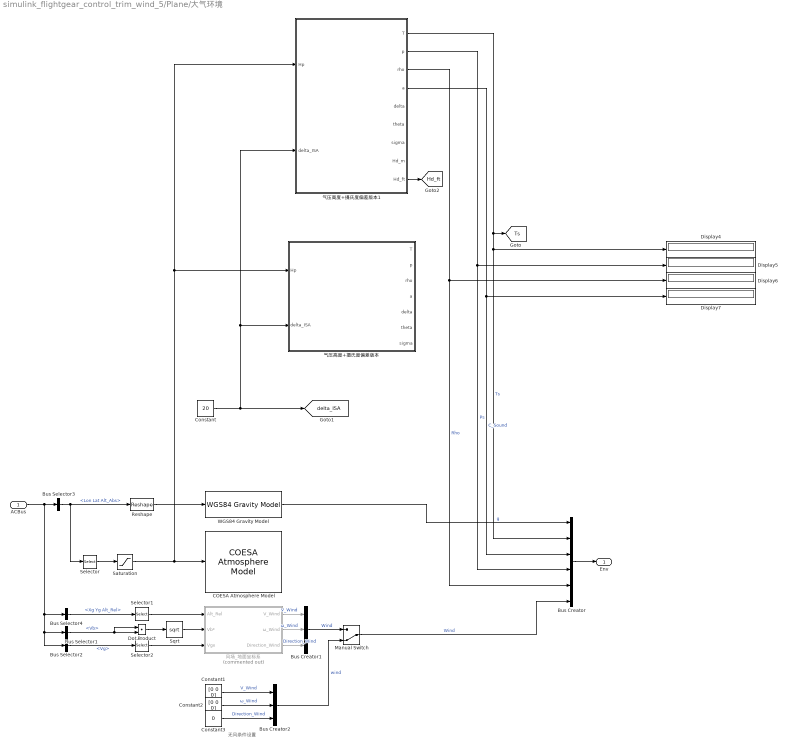
== system simulink_flightgear_control_trim_wind_5/Plane/大气环境 ==
  note: 无风条件设置
  ACBus : Inport
  Bus Creator : BusCreator  Inputs=6
  Bus Creator1 : BusCreator  Inputs=3
  Bus Creator2 : BusCreator  Inputs=3
  Bus Selector1 : BusSelector  OutputSignals=Vb
  Bus Selector2 : BusSelector  OutputSignals=Vg
  Bus Selector3 : BusSelector  OutputSignals=Lon Lat Alt_Abs
  Bus Selector4 : BusSelector  OutputSignals=Xg Yg Alt_Rel
  COESA Atmosphere Model : aerolibatmos2/COESA Atmosphere Model  units=Metric (MKS)  spec=1976 COESA-extended U.S. Standard Atmosphere  model=Profile  profile_var=High temperature  profile_percent=1%  profile_alt=5 km (16404 ft)  envelope_var=High temperature  envelope_percent=1%  action=Error
  Constant : Constant  Value=20
  Constant1 : Constant  Value=[0 0 0]
  Constant2 : Constant  Value=[0 0 0]
  Constant3 : Constant  Value=0
  Display{4..7} (4 alike) : Display
  Dot Product : DotProduct  OutDataTypeStr=double
  Manual Switch : ManualSwitch  CurrentSetting=0
  Reshape : Reshape  OutputDimensionality=Row vector (2-D)
  Saturation : Saturate  UpperLimit=84850  LowerLimit=1
  Selector : Selector  InputPortWidth=3  IndexOptions=Index vector (dialog)  Indices=[3]  OutputSizes=1
  Selector1 : Selector  InputPortWidth=3  IndexOptions=Index vector (dialog)  Indices=[3]  OutputSizes=1
  Selector2 : Selector  InputPortWidth=3  IndexOptions=Index vector (dialog)  Indices=[1]  OutputSizes=1
  Sqrt : Sqrt
  "WGS84 Gravity Model " : aerolibobsolete/WGS84 Gravity Model   model=WGS84 Taylor Series  units=Metric (MKS)  no_atmos=on  precessing=on  jd_loc=off  month=October  day=10  year=2004  no_centrifugal=on  action=None
  气压高度+摄氏度偏差版本 : MATLAB Function  TreatAsAtomicUnit=on
  气压高度+摄氏度偏差版本1 : MATLAB Function  TreatAsAtomicUnit=on
  风场_地面坐标系 : Subsystem  Commented=on
  Env : Outport  VectorParamsAs1DForOutWhenUnconnected=off
  tag scope: Hd_ft=global, Ts=global, delta_ISA=global
  wires:
  Bus Selector4/1 -> Selector1/1  "<Xg Yg Alt_Rel>"
  ACBus/1 -> Bus Selector2/1, Bus Selector1/1, Bus Selector4/1, Bus Selector3/1
  Bus Creator/1 -> Env/1
  气压高度+摄氏度偏差版本1/1(T) -> Bus Creator/2, Display4/1, [Ts]  "Ts"
  Selector1/1 -> 风场_地面坐标系/1(Alt_Rel)
  "WGS84 Gravity Model "/1 -> Bus Creator/1  "g"
  Bus Selector1/1 -> Dot Product/2, Dot Product/1  "<Vb>"
  Dot Product/1 -> Sqrt/1
  Sqrt/1 -> 风场_地面坐标系/2(Vb*)
  风场_地面坐标系/1(V_Wind) -> Bus Creator1/1  "V_Wind"
  风场_地面坐标系/2(ω_Wind) -> Bus Creator1/2  "ω_Wind"
  风场_地面坐标系/3(Direction_Wind) -> Bus Creator1/3  "Direction_Wind"
  Manual Switch/1 -> Bus Creator/6  "Wind"
  Bus Selector3/1 -> Reshape/1, Selector/1  "<Lon Lat Alt_Abs>"
  Reshape/1 -> "WGS84 Gravity Model "/1
  Bus Selector2/1 -> Selector2/1  "<Vg>"
  Selector2/1 -> 风场_地面坐标系/3(Vgx)
  Saturation/1 -> 气压高度+摄氏度偏差版本1/1(Hp), 气压高度+摄氏度偏差版本/1(Hp), COESA Atmosphere Model/1
  Bus Creator2/1 -> Manual Switch/2  "wind"
  Constant1/1 -> Bus Creator2/1  "V_Wind"
  Constant2/1 -> Bus Creator2/2  "ω_Wind"
  Bus Creator1/1 -> Manual Switch/1  "Wind"
  Constant3/1 -> Bus Creator2/3  "Direction_Wind"
  Selector/1 -> Saturation/1
  Constant/1 -> [delta_ISA], 气压高度+摄氏度偏差版本1/2(delta_ISA), 气压高度+摄氏度偏差版本/2(delta_ISA)
  气压高度+摄氏度偏差版本1/4(a) -> Bus Creator/3, Display7/1  "C_Sound"
  气压高度+摄氏度偏差版本1/3(rho) -> Bus Creator/5, Display6/1  "Rho"
  气压高度+摄氏度偏差版本1/2(p) -> Bus Creator/4, Display5/1  "Ps"
  气压高度+摄氏度偏差版本1/9(Hd_ft) -> [Hd_ft]

== system simulink_flightgear_control_trim_wind_5/Plane/气动力//力矩 ==
  Coefficients : Inport
  qbar : Inport  Port=2
  alpha : Inport  Port=3
  Demux : Demux  Outputs=3
  Demux1 : Demux  Outputs=[3,3]
      settings: DisplayOption=none
  Demux2 : Demux  Outputs=3
  Gain : Gain  Gain=[-1 1 -1]
  Gain1 : Gain  Gain=[1 1 1]
  MATLAB Function : MATLAB Function  TreatAsAtomicUnit=on
  Product : Product  InputSameDT=on  SaturateOnIntegerOverflow=on  OutDataTypeStr=Inherit: Same as first input
  Product3 : Product  InputSameDT=on  SaturateOnIntegerOverflow=on  OutDataTypeStr=Inherit: Same as first input
  Product4 : Product  Multiplication=Matrix(*)  RndMeth=Zero
  Radians to Degrees : simulink_extras/Transformations/Radians to Degrees
  Scope : Scope
  Scope1 : Scope
  reference area : Gain  Gain=Model.S  SaturateOnIntegerOverflow=on  OutDataTypeStr=Inherit: Same as input  ParamDataTypeStr=Inherit: Same as input
  reference length : Gain  Gain=[Model.b, Model.c, Model.b]  SaturateOnIntegerOverflow=on  OutDataTypeStr=Inherit: Same as input  ParamDataTypeStr=Inherit: Same as input
  Forces : Outport  VectorParamsAs1DForOutWhenUnconnected=off
  Moments : Outport  Port=2  VectorParamsAs1DForOutWhenUnconnected=off
  wires:
  reference length/1 -> Product3/2
  Coefficients/1 -> Demux1/1
  Demux1/2 -> Product3/1
  qbar/1 -> reference area/1
  reference area/1 -> reference length/1, Product/2
  Demux1/1 -> Gain/1
  Product3/1 -> Gain1/1
  Gain1/1 -> Demux/1, Moments/1
  Demux/2 -> Scope/1
  alpha/1 -> Radians to Degrees/1
  Radians to Degrees/1 -> MATLAB Function/1(u)
  MATLAB Function/1(y) -> Product4/1
  Product/1 -> Demux2/1, Forces/1
  Demux2/3 -> Scope1/1
  Gain/1 -> Product4/2
  Product4/1 -> Product/1

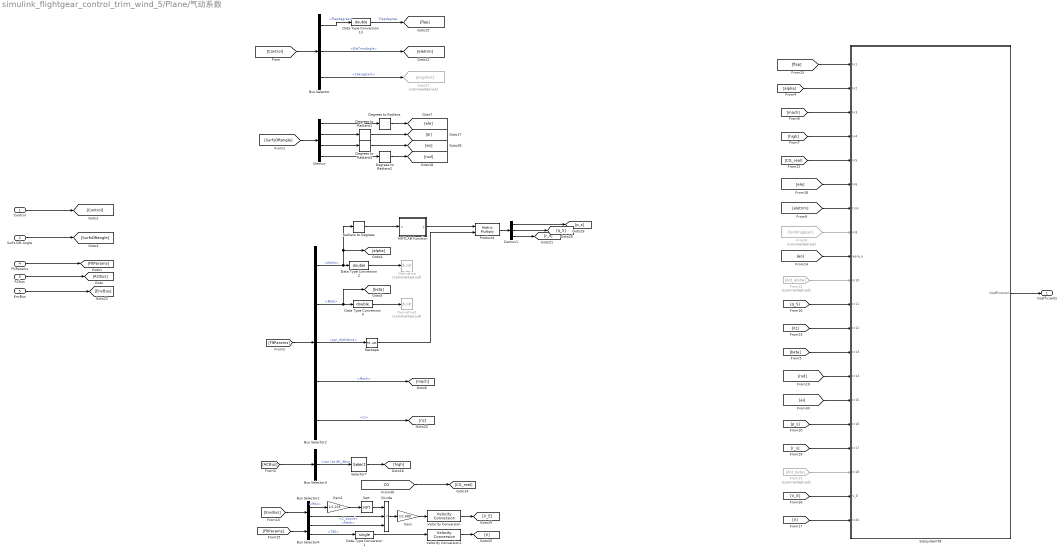
== system simulink_flightgear_control_trim_wind_5/Plane/气动系数 ==
  Control : Inport
  Surfs Dft Angle : Inport  Port=2
  ACbus : Inport  Port=3
  FltParams : Inport  Port=4
  EnvBus : Inport  Port=5
  Bus Selector : BusSelector  OutputSignals=Flapdegree,EleTrimAngle,10engstart
  Bus Selector1 : BusSelector  OutputSignals=Rho,C_Sound
  Bus Selector2 : BusSelector  OutputSignals=Alpha,Beta,pqr_WithWind,Mach,nz
  Bus Selector3 : BusSelector  OutputSignals=Lon Lat Alt_Abs
  Bus Selector4 : BusSelector  OutputSignals=Mach,TAS
  Data Type Conversion1 : DataTypeConversion  OutDataTypeStr=single  SaturateOnIntegerOverflow=off  RndMeth=Floor
  Data Type Conversion13 : DataTypeConversion  OutDataTypeStr=double  SaturateOnIntegerOverflow=off  RndMeth=Floor
  Data Type Conversion2 : DataTypeConversion  OutDataTypeStr=double  SaturateOnIntegerOverflow=off  RndMeth=Floor
  Data Type Conversion3 : DataTypeConversion  OutDataTypeStr=double  SaturateOnIntegerOverflow=off  RndMeth=Floor
  Degrees to Radians{,1..3} (4 alike) : simulink_extras/Transformations/Degrees to Radians
  Demux : Demux  Outputs=[1 2 2 1]
  Demux1 : Demux  Outputs=3
  Derivative : Derivative  Commented=on
  Derivative1 : Derivative  Commented=on
  Divide : Product  Inputs=***
  From12 : From  Commented=on  GotoTag=dot_alpha
  From13 : From  Commented=on  GotoTag=dot_beta
  From8 : From  Commented=on  GotoTag=landinggear
  Gain : Gain  Gain=1/1.689
  Gain1 : Gain  Gain=1/1.225
  Goto27 : Goto  Commented=on  GotoTag=engstart
  MATLAB Function : MATLAB Function  TreatAsAtomicUnit=on
  Product4 : Product  Multiplication=Matrix(*)  RndMeth=Zero
  Radians to Degrees : simulink_extras/Transformations/Radians to Degrees
  Reshape : Reshape  OutputDimensionality=Column vector (2-D)
  Selector7 : Selector  InputPortWidth=3  IndexOptions=Index vector (dialog)  Indices=[3]  OutputSizes=1
  Sqrt : Sqrt
  Subsystem58 : Subsystem
  Velocity Conversion : aerolibconvert2/Velocity Conversion  IU=m/s  OU=kts
  Velocity Conversion1 : aerolibconvert2/Velocity Conversion  IU=m/s  OU=kts
  Coefficients : Outport  VectorParamsAs1DForOutWhenUnconnected=off
  wires:
  [nz] -> Subsystem58/12(In12)
  Bus Selector2/4 -> [mach]  "<Mach>"
  [ele] -> Subsystem58/6(In6)
  Bus Selector2/3 -> Reshape/1  "<pqr_WithWind>"
  [p_s] -> Subsystem58/16(In16)
  [CG_real] -> Subsystem58/5(In5)
  Bus Selector/1 -> Data Type Conversion13/1  "<Flapdegree>"
  Bus Selector2/2 -> Data Type Conversion3/1, [beta]  "<Beta>"
  Subsystem58/1(Coefficients1) -> Coefficients/1
  [ACBus] -> Bus Selector3/1
  Bus Selector2/1 -> Radians to Degrees/1, [alpha], Data Type Conversion2/1  "<Alpha>"
  [rud] -> Subsystem58/14(In14)
  [ai] -> Subsystem58/15(In15)
  From12/1 -> Subsystem58/10(In10)
  From8/1 -> Subsystem58/8(In8)
  [mach] -> Subsystem58/3(In3)
  Control/1 -> [Control]
  [FltParams] -> Bus Selector2/1
  [Control] -> Bus Selector/1
  [r_s] -> Subsystem58/17(In17)
  [q_S] -> Subsystem58/11(In11)
  FltParams/1 -> [FltParams]
  [flap] -> Subsystem58/1(In1)
  [alpha] -> Subsystem58/2(In2)
  From13/1 -> Subsystem58/18(In18)
  Surfs Dft Angle/1 -> [SurfsDftangle]
  [beta] -> Subsystem58/13(In13)
  ACbus/1 -> [ACBus]
  [high] -> Subsystem58/4(In4)
  Bus Selector3/1 -> Selector7/1  "<Lon Lat Alt_Abs>"
  Selector7/1 -> [high]
  Bus Selector2/5 -> [nz]  "<nz>"
  Radians to Degrees/1 -> MATLAB Function/1(u)
  MATLAB Function/1(y) -> Product4/1
  Reshape/1 -> Product4/2
  Product4/1 -> Demux1/1
  Demux1/1 -> [p_s]
  Demux1/3 -> [r_s]
  Bus Selector/2 -> [eletrim]  "<EleTrimAngle>"
  [eletrim] -> Subsystem58/7(trim)
  EnvBus/1 -> [EnvBus]
  [EnvBus] -> Bus Selector1/1
  [FltParams] -> Bus Selector4/1
  Bus Selector1/1 -> Gain1/1  "<Rho>"
  Sqrt/1 -> Divide/1
  Bus Selector4/1 -> Divide/3  "<Mach>"
  Bus Selector1/2 -> Divide/2  "<C_Sound>"
  Divide/1 -> Gain/1
  Gain/1 -> Velocity Conversion/1
  [V_E] -> Subsystem58/19(V_E)
  Gain1/1 -> Sqrt/1
  Velocity Conversion/1 -> [V_E]
  Bus Selector4/2 -> Data Type Conversion1/1  "<TAS>"
  Velocity Conversion1/1 -> [V]
  [V] -> Subsystem58/20(In20)
  [ao] -> Subsystem58/9(aere_o)
  Demux1/2 -> [q_S]
  Bus Selector/3 -> Goto27/1  "<10engstart>"
  Data Type Conversion13/1 -> [flap]  "Flapdegree"
  Data Type Conversion1/1 -> Velocity Conversion1/1
  Demux/4 -> Degrees to Radians2/1
  Demux/1 -> Degrees to Radians/1
  Demux/3 -> Degrees to Radians3/1
  [SurfsDftangle] -> Demux/1
  Degrees to Radians1/1 -> [ai]
  Degrees to Radians2/1 -> [rud]
  Demux/2 -> Degrees to Radians1/1
  Degrees to Radians3/1 -> [ao]
  Degrees to Radians/1 -> [ele]
  Data Type Conversion2/1 -> Derivative/1
  Data Type Conversion3/1 -> Derivative1/1
  [CG] -> [CG_real]

== system simulink_flightgear_control_trim_wind_5/Plane/重力  ==
  Mass : Inport
  g : Inport  Port=2
  DCMwe : Inport  Port=3
  Ground to Wind : Product  Multiplication=Matrix(*)  InputSameDT=on  SaturateOnIntegerOverflow=on  OutDataTypeStr=Inherit: Same as first input
  Product : Product
  Reshape : Reshape  OutputDimensionality=Column vector (2-D)
  F_G : Outport  VectorParamsAs1DForOutWhenUnconnected=off
  A_G : Outport  Port=2  VectorParamsAs1DForOutWhenUnconnected=off
  wires:
  Reshape/1 -> Ground to Wind/2
  g/1 -> Reshape/1
  DCMwe/1 -> Ground to Wind/1
  Mass/1 -> Product/1
  Ground to Wind/1 -> Product/2, A_G/1
  Product/1 -> F_G/1

== system simulink_flightgear_control_trim_wind_5/Plane/重量//惯量 ==
  1-D Lookup Table1 : Lookup_n-D  NumberOfTableDimensions=1  BreakpointsForDimension1=Model.Ixx(1,:)  Table=Model.Ixx(2,:)  InternalRulePriority=Speed  RndMeth=Simplest
  1-D Lookup Table2 : Lookup_n-D  NumberOfTableDimensions=1  BreakpointsForDimension1=Model.Iyy(1,:)  Table=Model.Iyy(2,:)  InternalRulePriority=Speed  RndMeth=Simplest
  1-D Lookup Table3 : Lookup_n-D  NumberOfTableDimensions=1  BreakpointsForDimension1=Model.Izz(1,:)  Table=Model.Izz(2,:)  InternalRulePriority=Speed  RndMeth=Simplest
  1-D Lookup Table4 : Lookup_n-D  NumberOfTableDimensions=1  BreakpointsForDimension1=Model.Ixz(1,:)  Table=Model.Ixz(2,:)  InternalRulePriority=Speed  RndMeth=Simplest
  Constant1 : Constant  Value=15
  Constant2 : Constant  Value=250000
  Constant5 : Constant  Value=300000
  Gain : Gain  Gain=9.8
  Gain{10..13} (4 alike) : Gain  Gain=1/1000
  Gain14 : Gain
  Gain{2,4,15,19} (4 alike) : Gain  Gain=2.204622621849
  Gain{3,5,16,20} (4 alike) : Gain  Gain=1/9.8
  Gain{6..9} (4 alike) : Gain  Gain=10^6*1.35581795
  MATLAB Function1 : MATLAB Function  TreatAsAtomicUnit=on
  GW : Outport  VectorParamsAs1DForOutWhenUnconnected=off
  Inertia : Outport  Port=2  VectorParamsAs1DForOutWhenUnconnected=off
  CG_real : Outport  Port=3  VectorParamsAs1DForOutWhenUnconnected=off
  tag scope: mass=global
  wires:
  Constant1/1 -> CG_real/1
  Gain8/1 -> MATLAB Function1/3(izz)
  1-D Lookup Table1/1 -> Gain6/1
  Gain6/1 -> MATLAB Function1/1(ixx)
  1-D Lookup Table2/1 -> Gain7/1
  Constant5/1 -> GW/1, [mass], Gain/1
  1-D Lookup Table4/1 -> Gain9/1
  Gain9/1 -> MATLAB Function1/4(ixz)
  1-D Lookup Table3/1 -> Gain8/1
  MATLAB Function1/1(y) -> Gain14/1
  Gain12/1 -> 1-D Lookup Table1/1
  Gain11/1 -> 1-D Lookup Table2/1
  Gain10/1 -> 1-D Lookup Table3/1
  Gain13/1 -> 1-D Lookup Table4/1
  Gain14/1 -> Inertia/1
  Gain7/1 -> MATLAB Function1/2(iyy)
  Gain19/1 -> Gain12/1
  Gain2/1 -> Gain11/1
  Gain4/1 -> Gain10/1
  Gain15/1 -> Gain13/1
  Gain20/1 -> Gain19/1
  Gain3/1 -> Gain2/1
  Gain5/1 -> Gain4/1
  Gain16/1 -> Gain15/1
  Gain/1 -> Gain20/1, Gain3/1, Gain16/1, Gain5/1

== system simulink_flightgear_control_trim_wind_5/Plane/参数计算/Subsystem1 ==
  Vb : Inport
  " " : Sqrt  AlgorithmType=Newton-Raphson
  Data Type Conversion : DataTypeConversion  OutDataTypeStr=single  SaturateOnIntegerOverflow=off  RndMeth=Floor
  Data Type Conversion1 : DataTypeConversion  OutDataTypeStr=single  SaturateOnIntegerOverflow=off  RndMeth=Floor
  Data Type Conversion2 : DataTypeConversion  OutDataTypeStr=double  SaturateOnIntegerOverflow=off  RndMeth=Floor
  Product : Product  Inputs=*/  SaturateOnIntegerOverflow=on  OutDataTypeStr=Inherit: Same as first input
  Saturation : Saturate  UpperLimit=inf  LowerLimit=0.0001  ZeroCross=off
  Subsystem : Subsystem
  Subsystem1 : Subsystem
  Subsystem2 : Subsystem
  Trigonometric Function1 : Trigonometry  Operator=atan2
  Trigonometric Function2 : Trigonometry  Operator=asin
  Alpha : Outport  Unit=rad  InitialOutput=0  VectorParamsAs1DForOutWhenUnconnected=off
  Beta : Outport  Port=2  Unit=rad  InitialOutput=0  VectorParamsAs1DForOutWhenUnconnected=off
  V : Outport  Port=3  InitialOutput=0  VectorParamsAs1DForOutWhenUnconnected=off
  wires:
  Subsystem2/1(u²+v²+w²) -> " "/1
  Subsystem1/1(v) -> Product/1
  Vb/1 -> Subsystem/1(Vb), Subsystem1/1(Vb), Subsystem2/1(Vb)
  " "/1 -> V/1, Saturation/1
  Saturation/1 -> Product/2
  Subsystem/1(w) -> Trigonometric Function1/1
  Trigonometric Function1/1 -> Data Type Conversion/1
  Subsystem/2(u) -> Trigonometric Function1/2
  Data Type Conversion/1 -> Alpha/1
  Product/1 -> Data Type Conversion1/1
  Data Type Conversion1/1 -> Trigonometric Function2/1
  Trigonometric Function2/1 -> Data Type Conversion2/1
  Data Type Conversion2/1 -> Beta/1

== system simulink_flightgear_control_trim_wind_5/Plane/参数计算/qbar ==
  V_air : Inport
  rho : Inport  Port=2
  Constant : Constant  Value=0.5
  Product : Product  Inputs=3
  Product1 : Product
  qbar : Outport  VectorParamsAs1DForOutWhenUnconnected=off
  wires:
  Product/1 -> qbar/1
  rho/1 -> Product/1
  V_air/1 -> Product1/1, Product1/2
  Product1/1 -> Product/3
  Constant/1 -> Product/2

== system simulink_flightgear_control_trim_wind_5/Plane/参数计算/航迹角 ==
  Vg : Inport
  " " : Sqrt  AlgorithmType=Newton-Raphson
  Compare To Constant : simulink/Logic and Bit Operations/Compare To Constant  relop=>  const=0.1  OutDataTypeStr=boolean
  Product2 : Product
  Subsystem : Subsystem
  Subsystem1 : Subsystem
  Subsystem3 : Subsystem
  Trigonometric Function : Trigonometry  Operator=atan2
  Trigonometric Function1 : Trigonometry  Operator=atan2
  Unary Minus : UnaryMinus
  X : Outport  Unit=rad  InitialOutput=0  VectorParamsAs1DForOutWhenUnconnected=off
  Y : Outport  Port=2  Unit=rad  InitialOutput=0  VectorParamsAs1DForOutWhenUnconnected=off
  wires:
  Product2/1 -> Y/1
  Compare To Constant/1 -> Product2/2
  Trigonometric Function/1 -> X/1
  Trigonometric Function1/1 -> Product2/1
  Subsystem1/1(Vz) -> Unary Minus/1
  Unary Minus/1 -> Trigonometric Function1/1
  " "/1 -> Compare To Constant/1, Trigonometric Function1/2
  Subsystem/2(Vx) -> Trigonometric Function/2
  Subsystem3/1(Vx²+Vy²) -> " "/1
  Vg/1 -> Subsystem/1(Vg), Subsystem3/1(Vg), Subsystem1/1(Vg)
  Subsystem/1(Vy) -> Trigonometric Function/1

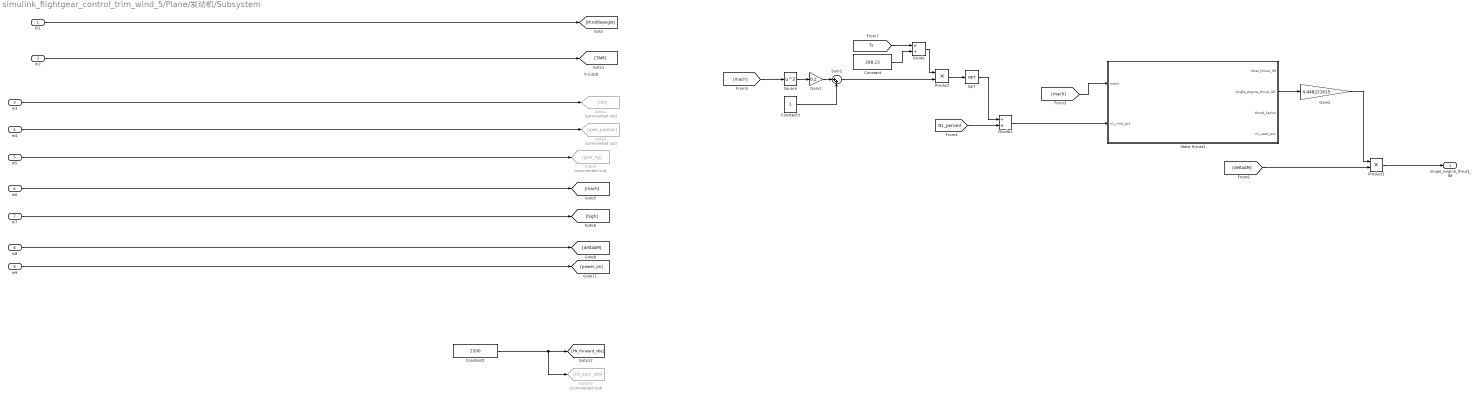
== system simulink_flightgear_control_trim_wind_5/Plane/发动机/Subsystem ==
  note: 华氏温度
  In1 : Inport
  In2 : Inport  Port=2
  In3 : Inport  Port=3
  In4 : Inport  Port=4
  In5 : Inport  Port=5
  In6 : Inport  Port=6
  In7 : Inport  Port=7
  In8 : Inport  Port=8
  In9 : Inport  Port=9
  Constant : Constant  Value=288.15
  Constant2 : Constant  Value=2500
  Constant3 : Constant
  Divide : Product  Inputs=*/
  Divide1 : Product  Inputs=/*
  Gain1 : Gain  Gain=0.2
  Gain2 : Gain  Gain=4.448221615
  Goto13 : Goto  Commented=on  GotoTag=FN_back_idle
  Goto2 : Goto  Commented=on  GotoTag=site
  Goto3 : Goto  Commented=on  GotoTag=gear_position
  Goto4 : Goto  Commented=on  GotoTag=gear_hg
  Product : Product
  Product1 : Product
  Sqrt : Sqrt
  Square : Math  Operator=square
  Static thrust1 : MATLAB Function  TreatAsAtomicUnit=on
  Sum2 : Sum  Inputs=|++
  single_engine_thrust_lbf : Outport
  wires:
  In2/1 -> [TAM]
  In1/1 -> [throttleangle]
  In5/1 -> Goto4/1
  In3/1 -> Goto2/1
  In4/1 -> Goto3/1
  In6/1 -> [mach]
  In8/1 -> [deltaAM]
  In7/1 -> [high]
  In9/1 -> [power_on]
  Constant2/1 -> [FN_forward_idle], Goto13/1
  Product1/1 -> single_engine_thrust_lbf/1
  Divide1/1 -> Static thrust1/2(n1_cmd_pct)
  [mach] -> Static thrust1/1(mach)
  Sqrt/1 -> Divide1/1
  [N1_percent] -> Divide1/2
  Product/1 -> Sqrt/1
  Constant3/1 -> Sum2/2
  [Ts] -> Divide/1
  Sum2/1 -> Product/2
  Gain1/1 -> Sum2/1
  Constant/1 -> Divide/2
  [mach] -> Square/1
  Square/1 -> Gain1/1
  Divide/1 -> Product/1
  [deltaAM] -> Product1/2
  Static thrust1/2(single_engine_thrust_lbf) -> Gain2/1
  Gain2/1 -> Product1/1

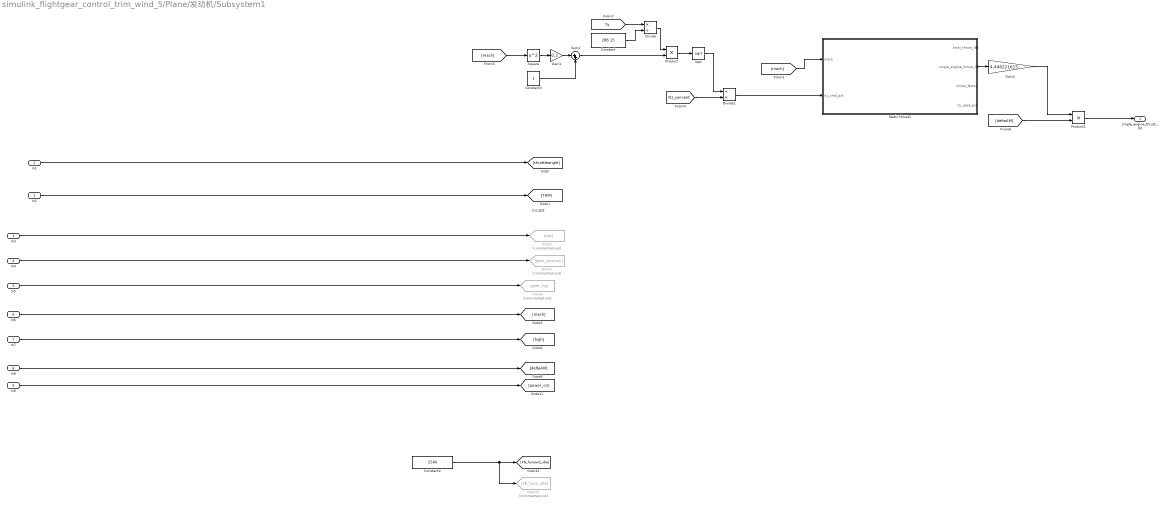
== system simulink_flightgear_control_trim_wind_5/Plane/发动机/Subsystem1 ==
  note: 华氏温度
  In1 : Inport
  In2 : Inport  Port=2
  In3 : Inport  Port=3
  In4 : Inport  Port=4
  In5 : Inport  Port=5
  In6 : Inport  Port=6
  In7 : Inport  Port=7
  In8 : Inport  Port=8
  In9 : Inport  Port=9
  Constant : Constant  Value=288.15
  Constant2 : Constant  Value=2500
  Constant3 : Constant
  Divide : Product  Inputs=*/
  Divide1 : Product  Inputs=/*
  Gain1 : Gain  Gain=0.2
  Gain2 : Gain  Gain=4.448221615
  Goto13 : Goto  Commented=on  GotoTag=FN_back_idle
  Goto2 : Goto  Commented=on  GotoTag=site
  Goto3 : Goto  Commented=on  GotoTag=gear_position
  Goto4 : Goto  Commented=on  GotoTag=gear_hg
  Product : Product
  Product1 : Product
  Sqrt : Sqrt
  Square : Math  Operator=square
  Static thrust1 : MATLAB Function  TreatAsAtomicUnit=on
  Sum2 : Sum  Inputs=|++
  single_engine_thrust_lbf : Outport
  wires:
  In2/1 -> [TAM]
  In1/1 -> [throttleangle]
  In5/1 -> Goto4/1
  In3/1 -> Goto2/1
  In4/1 -> Goto3/1
  In6/1 -> [mach]
  In8/1 -> [deltaAM]
  In7/1 -> [high]
  In9/1 -> [power_on]
  Constant2/1 -> [FN_forward_idle], Goto13/1
  Product1/1 -> single_engine_thrust_lbf/1
  [N1_percent] -> Divide1/2
  Divide1/1 -> Static thrust1/2(n1_cmd_pct)
  Divide/1 -> Product/1
  [mach] -> Square/1
  [Ts] -> Divide/1
  Constant3/1 -> Sum2/2
  [mach] -> Static thrust1/1(mach)
  Constant/1 -> Divide/2
  Gain1/1 -> Sum2/1
  Sum2/1 -> Product/2
  Square/1 -> Gain1/1
  Sqrt/1 -> Divide1/1
  Product/1 -> Sqrt/1
  [deltaAM] -> Product1/2
  Static thrust1/2(single_engine_thrust_lbf) -> Gain2/1
  Gain2/1 -> Product1/1

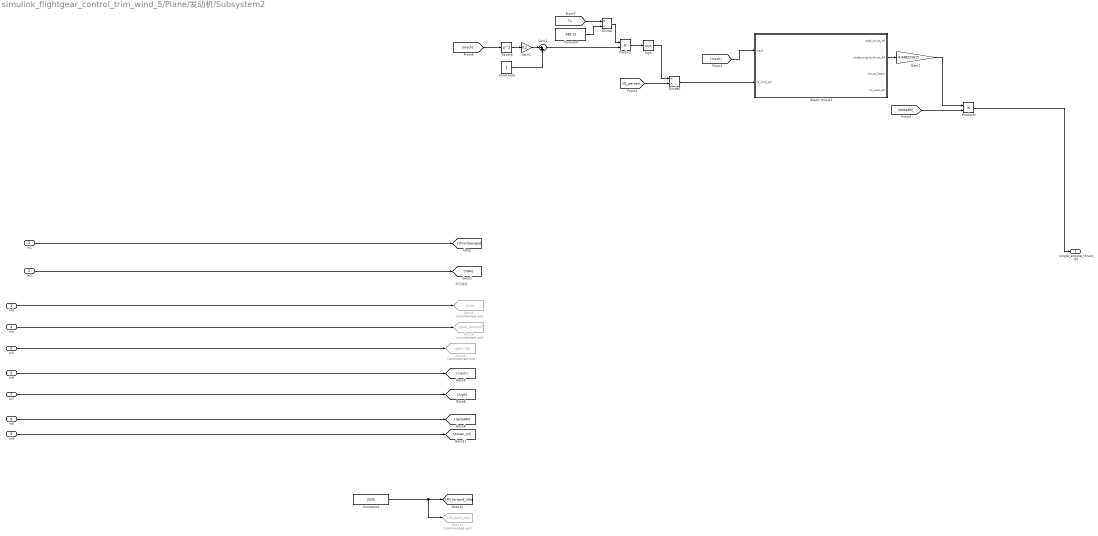
== system simulink_flightgear_control_trim_wind_5/Plane/发动机/Subsystem2 ==
  note: 华氏温度
  In1 : Inport
  In2 : Inport  Port=2
  In3 : Inport  Port=3
  In4 : Inport  Port=4
  In5 : Inport  Port=5
  In6 : Inport  Port=6
  In7 : Inport  Port=7
  In8 : Inport  Port=8
  In9 : Inport  Port=9
  Constant : Constant  Value=288.15
  Constant2 : Constant  Value=2500
  Constant3 : Constant
  Divide : Product  Inputs=*/
  Divide1 : Product  Inputs=/*
  Gain1 : Gain  Gain=0.2
  Gain2 : Gain  Gain=4.448221615
  Goto13 : Goto  Commented=on  GotoTag=FN_back_idle
  Goto2 : Goto  Commented=on  GotoTag=site
  Goto3 : Goto  Commented=on  GotoTag=gear_position
  Goto4 : Goto  Commented=on  GotoTag=gear_hg
  Product : Product
  Product1 : Product
  Sqrt : Sqrt
  Square : Math  Operator=square
  Static thrust1 : MATLAB Function  TreatAsAtomicUnit=on
  Sum2 : Sum  Inputs=|++
  single_engine_thrust_lbf : Outport
  wires:
  In2/1 -> [TAM]
  In1/1 -> [throttleangle]
  In5/1 -> Goto4/1
  In3/1 -> Goto2/1
  In4/1 -> Goto3/1
  In6/1 -> [mach]
  In8/1 -> [deltaAM]
  In7/1 -> [high]
  In9/1 -> [power_on]
  Constant2/1 -> [FN_forward_idle], Goto13/1
  Product1/1 -> single_engine_thrust_lbf/1
  [N1_percent] -> Divide1/2
  Divide1/1 -> Static thrust1/2(n1_cmd_pct)
  Divide/1 -> Product/1
  [mach] -> Square/1
  [Ts] -> Divide/1
  Constant3/1 -> Sum2/2
  [mach] -> Static thrust1/1(mach)
  Constant/1 -> Divide/2
  Gain1/1 -> Sum2/1
  Sum2/1 -> Product/2
  Square/1 -> Gain1/1
  Sqrt/1 -> Divide1/1
  Product/1 -> Sqrt/1
  [deltaAM] -> Product1/2
  Static thrust1/2(single_engine_thrust_lbf) -> Gain2/1
  Gain2/1 -> Product1/1
